simulink model "SimulaVelocidad_alumnos"  (R2024b)
settings: Solver=VariableStepAuto  StartTime=0.0  StopTime=30  FixedStep=0.02  MaxStep=0.02  RelTol=1e-6
values from neighbouring files (symbols this model uses):
  D = 0.074118    [Ensayo K250 17_42.mat]    (also in parametros_6_1.m)
  K = 125    [Ensayo K250 17_42.mat]    (also in EnsayoRobot.m = 8.25082508251; parametros_6_1.m = 107.5)
  Km = 0.0020745    [Ensayo K250 17_42.mat]    (also in parametros_6_1.m)
  Tm = 0.061095    [Ensayo K250 17_42.mat]    (also in parametros_6_1.m)
settings Model: Creator=stic  LastModifiedBy=Usuario
settings DataIOCC: ReturnWorkspaceOutputs=off
settings RTWCC: GPUComputeCapability=3.5

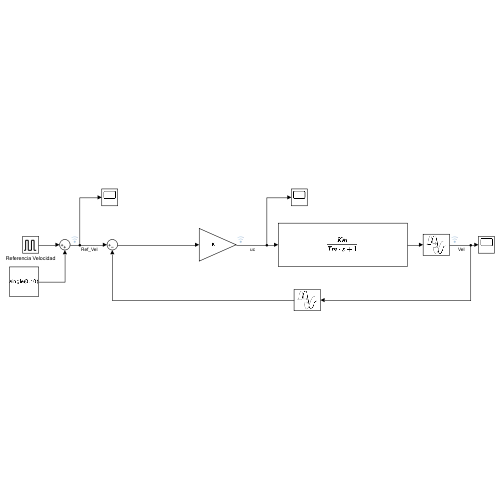
[thumbnail: Simulink's stored preview of the top-level diagram]
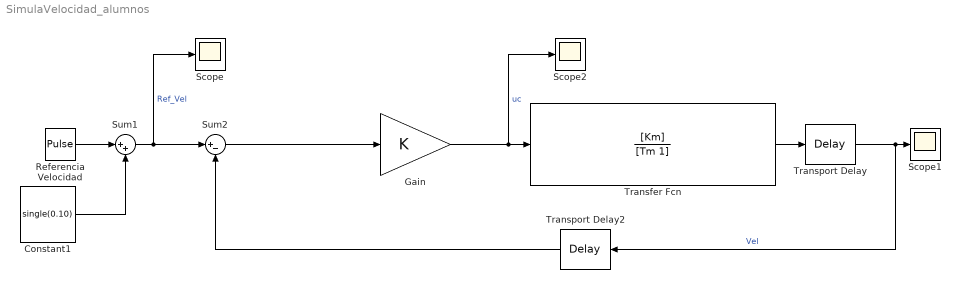
== system SimulaVelocidad_alumnos ==
  Constant1 : Constant  Value=single(0.10)
  Gain : Gain  Gain=K
  Referencia Velocidad : DiscretePulseGenerator  PulseType=Time based  Amplitude=single(0.05)  Period=10  PulseWidth=50  PhaseDelay=5  SampleTime=500
  Scope : Scope
  Scope1 : Scope
  Scope2 : Scope
  Sum1 : Sum  Inputs=|++
  Sum2 : Sum  Inputs=|+-
  Transfer Fcn : TransferFcn  Numerator=[Km]  Denominator=[Tm 1]
  Transport Delay : TransportDelay  DelayTime=D
  Transport Delay2 : TransportDelay  DelayTime=0.02/2
  wires:
  Transfer Fcn/1 -> Transport Delay/1
  Referencia Velocidad/1 -> Sum1/1
  Constant1/1 -> Sum1/2
  Gain/1 -> Transfer Fcn/1, Scope2/1  "uc"
  Sum1/1 -> Scope/1, Sum2/1  "Ref_Vel"
  Transport Delay/1 -> Scope1/1, Transport Delay2/1  "Vel"
  Sum2/1 -> Gain/1
  Transport Delay2/1 -> Sum2/2
